simulink model "single_phase_ttype_inverter"  (R2026a)
settings: Solver=ode23tb  StopTime=simlength  FixedStep=tc  MaxStep=glb_time.tc
values from neighbouring files (symbols this model uses):
  afe_ctrl = param.afe.ctrl    [init_model.m]
  afe_pwm_phase_shift_mod1 = param.afe.behav.pwm_phase_shift_mod1    [init_model.m]
  DThs_init = param.thermal.DThs_init    [init_model.m]
  filters = param.ctrl.filters    [init_model.m]
  frt_data = param.frt.data    [init_model.m]
  glb_time = param.glb_time    [init_model.m]
  grid_emu = param.grid.emu    [init_model.m]
  kepsilon = param.spinv.kepsilon    [init_model.m]
  kp_align = param.ctrl.kp_align    [init_model.m]
  lim_down_align = param.ctrl.lim_down_align    [init_model.m]
  lim_up_align = param.ctrl.lim_up_align    [init_model.m]
  mavarage_filter_frequency_base_order = param.ctrl.mavarage_filter_frequency_base_order    [init_model.m]
  omega_set = param.spinv.omega_set    [init_model.m]
  single_phase_inverter_ctrl = param.spinv.ctrl    [init_model.m]
  Tambient = param.thermal.Tambient    [init_model.m]
  time_aux_power_supply_fault = param.sim.time_aux_power_supply_fault    [init_model.m]
  time_step_ref_1 = param.spinv.ref.time_step_ref_1    [init_model.m]
  time_step_ref_2 = param.spinv.ref.time_step_ref_2    [init_model.m]
  time_step_ref_3 = param.spinv.ref.time_step_ref_3    [init_model.m]
undefined symbols (not defined in the file or in its folder): delta_fht1, hwdata, ki_align, Ld_fht1, magnitude, omega_fht1, ts_inv, Vac_FS, Vdc_nom, Xbez
libraries: fl_lib x61, nesl_utility x39, moving_average_filter x11, moving_average_filter_cc x8, discrete_time_low_pass_filter x4, sl_discontinuities x3, single_phase_transformer_lib x3, linear_double_integrator_observer_ccaller x2, phase_shift_filter_ccaller x2, threephase_inductor_lib x1, dclink_for_two_levels x1, three_phase_pwm_modulator x1
(part 8 of 9)

== system single_phase_ttype_inverter/afe/AFE_control/afe_control/grid_voltage_phase_lock_loops/dq_pll/pll_stageB/double_integrator_observer ==
  phase : Inport
  Gain : Gain  Gain=afe_ctrl.di_obs.Ldso  Multiplication=Matrix(K*u)
  Gain1 : Gain  Gain=afe_ctrl.di_obs.Adso  Multiplication=Matrix(K*u)
  Gain2 : Gain  Gain=afe_ctrl.di_obs.Cso  Multiplication=Matrix(K*u)
  Selector : Selector  InputPortWidth=2  IndexOptions=Index vector (dialog)  Indices=2  OutputSizes=1
  Sum : Sum  Inputs=-+|
  Sum1 : Sum  Inputs=|++
  Unit Delay : UnitDelay  SampleTime=-1
  bounder1 : MATLAB Function  TreatAsAtomicUnit=on
  bounder2 : MATLAB Function  TreatAsAtomicUnit=on
  omega_hat : Outport
  wires:
  Gain/1 -> Sum1/1
  Selector/1 -> omega_hat/1
  Gain2/1 -> bounder2/1(u)  "theta_hat"
  Gain1/1 -> Sum1/2
  Sum1/1 -> Unit Delay/1
  Sum/1 -> bounder1/1(u)  "e"
  Unit Delay/1 -> Gain1/1, Selector/1, Gain2/1
  phase/1 -> Sum/2  "phase"
  bounder1/1(y) -> Gain/1  "e_bounded"
  bounder2/1(y) -> Sum/1  "theta_hat_bounded"

== system single_phase_ttype_inverter/afe/AFE_control/afe_control/grid_voltage_phase_lock_loops/dq_pll/pll_stageB/scheduled-p-gain ==
  In1 : Inport
  Switch : Switch  Criteria=u2 > Threshold  Threshold=0.5  SaturateOnIntegerOverflow=off  InputSameDT=off
  kp1 : Gain  Gain=afe_ctrl.pll_p  SaturateOnIntegerOverflow=on  OutDataTypeStr=Inherit: Same as input  ParamDataTypeStr=Inherit: Same as input
  kp3 : Gain  Gain=afe_ctrl.pll_p_frt  SaturateOnIntegerOverflow=on  OutDataTypeStr=Inherit: Same as input  ParamDataTypeStr=Inherit: Same as input
  Out2 : Outport
  wires:
  kp3/1 -> Switch/1
  kp1/1 -> Switch/3
  [frt_active_mod1] -> Switch/2
  In1/1 -> kp1/1, kp3/1
  Switch/1 -> Out2/1

== system single_phase_ttype_inverter/single_phase_inverter/single phase inverter control/single_phase_inverter_ctrl/single_phase_current_control/dqpi_current_controller/dq_vector_pi_ccaller/Reset ==
  Step : Step  Time=0.05  InitialValue=1  FinalValue=0
  en : Outport
  wires:
  Step/1 -> en/1

== system single_phase_ttype_inverter/single_phase_inverter/single phase inverter control/single_phase_inverter_ctrl/single_phase_current_control/dqpi_current_controller/i2alphabeta/first_harmonic_tracker ==
  u : Inport
  Bus Selector : BusSelector  OutputSignals=output_pu_hat,output_pu_hat_dot
  Constant1 : Constant  Value=6
  Constant2 : Constant  Value=glb_time.ts_inv
  Constant3 : Constant  Value=single_phase_inverter_ctrl.fht_load.omega_fht
  Constant4 : Constant  Value=single_phase_inverter_ctrl.fht_load.delta_fht
  Constant5 : Constant  Value=single_phase_inverter_ctrl.fht_load.Ld_fht(1)
  Constant6 : Constant  Value=single_phase_inverter_ctrl.fht_load.Ld_fht(2)
  Data Type Conversion{1..2,6..9} (6 alike) : DataTypeConversion  OutDataTypeStr=single  SaturateOnIntegerOverflow=off  RndMeth=Floor
  Data Type Conversion10 : DataTypeConversion  OutDataTypeStr=double  SaturateOnIntegerOverflow=off  RndMeth=Floor
  Data Type Conversion3 : DataTypeConversion  OutDataTypeStr=uint8  SaturateOnIntegerOverflow=off  RndMeth=Floor
  Data Type Conversion4 : DataTypeConversion  OutDataTypeStr=double  SaturateOnIntegerOverflow=off  RndMeth=Floor
  Data Type Conversion5 : DataTypeConversion  OutDataTypeStr=uint8  SaturateOnIntegerOverflow=off  RndMeth=Floor
  Gain : Gain  Gain=-1/single_phase_inverter_ctrl.fht_load.omega_fht
  Step : Step  Time=0.0125  InitialValue=1  FinalValue=0
  first_harmonic_tracker : CCaller  FunctionName=first_harmonic_tracker_process_simulink  PortSpecificationStruct="%)30     .    B \\   8    (     @         %    \"     D    !     0         %  0 \"0    $    _    07)G3F%M90  4&]R=$YA;64 4V-O<&4     26YD97@     5'EP90      4VEZ90      27-';&]B86P   X    P    !@    @    $          4    (     0    ,    !         !   P!O=70 #@   #     &    \"     0         !0    @    !     P    $         $  # &]U=  .    .     8    (    !          %    \"     $    &     0         0  ...(+4988 chars)"
  alpha : Outport
  beta : Outport  Port=2
  wires:
  Data Type Conversion4/1 -> alpha/1
  Data Type Conversion3/1 -> first_harmonic_tracker/1
  Data Type Conversion1/1 -> first_harmonic_tracker/3
  Data Type Conversion2/1 -> first_harmonic_tracker/2
  first_harmonic_tracker/1 -> Bus Selector/1
  Bus Selector/1 -> Data Type Conversion4/1  "<output_pu_hat>"
  Step/1 -> Data Type Conversion3/1
  u/1 -> Data Type Conversion2/1
  Constant2/1 -> Data Type Conversion1/1
  Constant1/1 -> Data Type Conversion5/1
  Data Type Conversion5/1 -> first_harmonic_tracker/8
  Constant3/1 -> Data Type Conversion6/1
  Data Type Conversion6/1 -> first_harmonic_tracker/4
  Constant4/1 -> Data Type Conversion7/1
  Data Type Conversion7/1 -> first_harmonic_tracker/5
  Constant5/1 -> Data Type Conversion8/1
  Data Type Conversion8/1 -> first_harmonic_tracker/6
  Constant6/1 -> Data Type Conversion9/1
  Data Type Conversion9/1 -> first_harmonic_tracker/7
  Bus Selector/2 -> Data Type Conversion10/1  "<output_pu_hat_dot>"
  Data Type Conversion10/1 -> Gain/1
  Gain/1 -> beta/1

== system single_phase_ttype_inverter/single_phase_inverter/single phase inverter control/single_phase_inverter_ctrl/single_phase_current_control/dqpi_current_controller/i2alphabeta/phase_shift_method ==
  i_alpha : Inport
  Gain : Gain  Gain=-1
  phase shift filter : phase_shift_filter/phase shift filter  f=frequency_set  scaling_factor=1  ts=glb_time.ts_inv
  i_alpha_phase_shift_m : Outport
  i_beta_phase_shift_m : Outport  Port=2
  wires:
  i_alpha/1 -> phase shift filter/1, i_alpha_phase_shift_m/1
  Gain/1 -> i_beta_phase_shift_m/1  "i_beta_phase_shift_methos"
  phase shift filter/1 -> Gain/1

== system single_phase_ttype_inverter/single_phase_inverter/single phase inverter control/single_phase_inverter_ctrl/single_phase_current_control/dqpi_current_controller/i2alphabeta/phase_shift_method_ccaller ==
  i_alpha : Inport
  Gain : Gain  Gain=-1
  phase_shift_filter_ccaller : phase_shift_filter_ccaller/phase_shift_filter_ccaller  freq_m=frequency_set  ts_m=glb_time.ts_inv  scaling_m=1  reset_time_release=0.025  instance=0  tc_m=-1
  i_alpha_phase_shift_m : Outport
  i_beta_phase_shift_m : Outport  Port=2
  wires:
  phase_shift_filter_ccaller/1 -> Gain/1
  Gain/1 -> i_beta_phase_shift_m/1  "i_beta_phase_shift_methos"
  i_alpha/1 -> i_alpha_phase_shift_m/1, phase_shift_filter_ccaller/1

== system single_phase_ttype_inverter/single_phase_inverter/single phase inverter control/single_phase_inverter_ctrl/single_phase_current_control/dqpi_current_controller/i2alphabeta/sogi ==
  u : Inport
  Constant2 : Constant  Value=omega_set
  Product : Product
  Product1 : Product
  Sum1 : Sum  Inputs=|+-
  Sum3 : Sum  Inputs=-+|
  integrator_1 : Subsystem
  integrator_2 : Subsystem
  kepsilon : Gain  Gain=kepsilon
  ualpha : Outport
  ubeta : Outport  Port=2
  wires:
  u/1 -> ualpha/1, Sum3/2
  Sum3/1 -> kepsilon/1
  kepsilon/1 -> Sum1/1
  Sum1/1 -> Product/2
  Product/1 -> integrator_1/1(in)
  integrator_1/1(out) -> Product1/2, Sum3/1
  Constant2/1 -> Product/1, Product1/1
  Product1/1 -> integrator_2/1(in)
  integrator_2/1(out) -> ubeta/1, Sum1/2

== system single_phase_ttype_inverter/single_phase_inverter/single phase inverter control/single_phase_inverter_ctrl/single_phase_current_control/dqpi_current_controller/i2alphabeta/sogi_ccaller ==
  input : Inport
  Bus Selector : BusSelector  OutputSignals=sogi_flt_output_alpha,sogi_flt_output_beta
  CCaller : CCaller  FunctionName=sogi_flt_process_simulink  PortSpecificationStruct="%)30     .    . P   8    (     @         %    \"     <    !     0         %  0 \"0    $    _    07)G3F%M90  4&]R=$YA;64 4V-O<&4     26YD97@     5'EP90      4VEZ90      27-';&]B86P   X    P    !@    @    $          4    (     0    ,    !         !   P!O=70 #@   #     &    \"     0         !0    @    !     P    $         $  # &]U=  .    .     8    (    !          %    \"     $    &     0         0   ...(+3829 chars)"
  Constant1 : Constant  Value=glb_time.ts_inv
  Constant2 : Constant  Value=omega_set
  Constant3 : Constant  Value=kepsilon
  Constant4 : Constant  Value=2
  Data Type Conversion{1..2,4,6} (4 alike) : DataTypeConversion  OutDataTypeStr=single  SaturateOnIntegerOverflow=off  RndMeth=Floor
  Data Type Conversion3 : DataTypeConversion  OutDataTypeStr=uint8  SaturateOnIntegerOverflow=off  RndMeth=Floor
  Data Type Conversion5 : DataTypeConversion  OutDataTypeStr=double  SaturateOnIntegerOverflow=off  RndMeth=Floor
  Data Type Conversion7 : DataTypeConversion  OutDataTypeStr=double  SaturateOnIntegerOverflow=off  RndMeth=Floor
  Data Type Conversion8 : DataTypeConversion  OutDataTypeStr=uint8  SaturateOnIntegerOverflow=off  RndMeth=Floor
  Reset : Subsystem
  Terminator : Terminator
  Zero-Order Hold{1..6} (6 alike) : ZeroOrderHold  SampleTime=-1
  alpha : Outport
  beta : Outport  Port=2
  wires:
  Zero-Order Hold6/1 -> Data Type Conversion4/1
  Data Type Conversion4/1 -> CCaller/1
  Bus Selector/1 -> Data Type Conversion7/1  "<sogi_flt_output_alpha>"
  CCaller/1 -> Bus Selector/1
  Constant4/1 -> Zero-Order Hold5/1
  Zero-Order Hold5/1 -> Data Type Conversion3/1
  Constant2/1 -> Zero-Order Hold1/1
  Zero-Order Hold1/1 -> Data Type Conversion2/1
  Zero-Order Hold2/1 -> Data Type Conversion1/1
  Constant1/1 -> Zero-Order Hold2/1
  Reset/1(en) -> Zero-Order Hold4/1
  Zero-Order Hold4/1 -> Data Type Conversion8/1
  input/1 -> alpha/1, Zero-Order Hold6/1
  Bus Selector/2 -> Data Type Conversion5/1  "<sogi_flt_output_beta>"
  Data Type Conversion5/1 -> beta/1
  Data Type Conversion3/1 -> CCaller/6
  Data Type Conversion8/1 -> CCaller/5
  Data Type Conversion2/1 -> CCaller/3
  Data Type Conversion1/1 -> CCaller/2
  Data Type Conversion6/1 -> CCaller/4
  Zero-Order Hold3/1 -> Data Type Conversion6/1
  Constant3/1 -> Zero-Order Hold3/1
  Data Type Conversion7/1 -> Terminator/1

== system single_phase_ttype_inverter/single_phase_inverter/single phase inverter control/single_phase_inverter_ctrl/sistem_identification/open loop u//f/sogi_ccaller/Reset ==
  Step : Step  Time=0.025  InitialValue=1  FinalValue=0
  en : Outport
  wires:
  Step/1 -> en/1

== system single_phase_ttype_inverter/afe/AFE_control/afe_control/grid_voltage_phase_lock_loops/DDSRF-PLL/pll_stageA/filter_and_transformation/first_harmonic_tracker_phase_u ==
  u : Inport
  Bus Selector : BusSelector  OutputSignals=output_pu_hat
  C Caller : CCaller  FunctionName=first_harmonic_tracker_process_simulink  PortSpecificationStruct="%)30     .    B \\   8    (     @         %    \"     D    !     0         %  0 \"0    $    _    07)G3F%M90  4&]R=$YA;64 4V-O<&4     26YD97@     5'EP90      4VEZ90      27-';&]B86P   X    P    !@    @    $          4    (     0    ,    !         !   P!O=70 #@   #     &    \"     0         !0    @    !     P    $         $  # &]U=  .    .     8    (    !          %    \"     $    &     0         0  ...(+4988 chars)"
  Constant : Constant  Value=glb_time.ts_afe
  Constant1 : Constant  Value=6
  Constant4 : Constant  Value=afe_ctrl.fht_grid.omega_fht
  Constant5 : Constant  Value=afe_ctrl.fht_grid.delta_fht
  Constant6 : Constant  Value=afe_ctrl.fht_grid.Ld_fht(1)
  Constant7 : Constant  Value=afe_ctrl.fht_grid.Ld_fht(2)
  Data Type Conversion{1..2,6..9} (6 alike) : DataTypeConversion  OutDataTypeStr=single  SaturateOnIntegerOverflow=off  RndMeth=Floor
  Data Type Conversion3 : DataTypeConversion  OutDataTypeStr=uint8  SaturateOnIntegerOverflow=off  RndMeth=Floor
  Data Type Conversion4 : DataTypeConversion  OutDataTypeStr=double  SaturateOnIntegerOverflow=off  RndMeth=Floor
  Data Type Conversion5 : DataTypeConversion  OutDataTypeStr=uint8  SaturateOnIntegerOverflow=off  RndMeth=Floor
  Step : Step  Time=0.0125  InitialValue=1  FinalValue=0
  u_hat : Outport
  wires:
  Data Type Conversion4/1 -> u_hat/1
  Data Type Conversion3/1 -> C Caller/1
  Data Type Conversion1/1 -> C Caller/3
  Data Type Conversion2/1 -> C Caller/2
  C Caller/1 -> Bus Selector/1
  Bus Selector/1 -> Data Type Conversion4/1  "<output_pu_hat>"
  Step/1 -> Data Type Conversion3/1
  u/1 -> Data Type Conversion2/1
  Constant/1 -> Data Type Conversion1/1
  Constant1/1 -> Data Type Conversion5/1
  Constant4/1 -> Data Type Conversion6/1
  Constant6/1 -> Data Type Conversion8/1
  Constant7/1 -> Data Type Conversion9/1
  Constant5/1 -> Data Type Conversion7/1
  Data Type Conversion5/1 -> C Caller/8
  Data Type Conversion6/1 -> C Caller/4
  Data Type Conversion7/1 -> C Caller/5
  Data Type Conversion8/1 -> C Caller/6
  Data Type Conversion9/1 -> C Caller/7

== system single_phase_ttype_inverter/afe/AFE_control/afe_control/grid_voltage_phase_lock_loops/DDSRF-PLL/pll_stageA/filter_and_transformation/first_harmonic_tracker_phase_v ==
  u : Inport
  Bus Selector : BusSelector  OutputSignals=output_pu_hat
  C Caller : CCaller  FunctionName=first_harmonic_tracker_process_simulink  PortSpecificationStruct="%)30     .    B \\   8    (     @         %    \"     D    !     0         %  0 \"0    $    _    07)G3F%M90  4&]R=$YA;64 4V-O<&4     26YD97@     5'EP90      4VEZ90      27-';&]B86P   X    P    !@    @    $          4    (     0    ,    !         !   P!O=70 #@   #     &    \"     0         !0    @    !     P    $         $  # &]U=  .    .     8    (    !          %    \"     $    &     0         0  ...(+4988 chars)"
  Constant : Constant  Value=glb_time.ts_afe
  Constant1 : Constant  Value=8
  Constant4 : Constant  Value=afe_ctrl.fht_grid.omega_fht
  Constant5 : Constant  Value=afe_ctrl.fht_grid.delta_fht
  Constant6 : Constant  Value=afe_ctrl.fht_grid.Ld_fht(1)
  Constant7 : Constant  Value=afe_ctrl.fht_grid.Ld_fht(2)
  Data Type Conversion{1..2,6..9} (6 alike) : DataTypeConversion  OutDataTypeStr=single  SaturateOnIntegerOverflow=off  RndMeth=Floor
  Data Type Conversion3 : DataTypeConversion  OutDataTypeStr=uint8  SaturateOnIntegerOverflow=off  RndMeth=Floor
  Data Type Conversion4 : DataTypeConversion  OutDataTypeStr=double  SaturateOnIntegerOverflow=off  RndMeth=Floor
  Data Type Conversion5 : DataTypeConversion  OutDataTypeStr=uint8  SaturateOnIntegerOverflow=off  RndMeth=Floor
  Step : Step  Time=0.0125  InitialValue=1  FinalValue=0
  u_hat : Outport
  wires:
  Data Type Conversion9/1 -> C Caller/7
  Data Type Conversion8/1 -> C Caller/6
  Data Type Conversion7/1 -> C Caller/5
  Data Type Conversion6/1 -> C Caller/4
  Data Type Conversion5/1 -> C Caller/8
  Constant5/1 -> Data Type Conversion7/1
  Constant7/1 -> Data Type Conversion9/1
  Constant6/1 -> Data Type Conversion8/1
  Constant4/1 -> Data Type Conversion6/1
  Constant1/1 -> Data Type Conversion5/1
  Constant/1 -> Data Type Conversion1/1
  u/1 -> Data Type Conversion2/1
  Step/1 -> Data Type Conversion3/1
  Bus Selector/1 -> Data Type Conversion4/1  "<output_pu_hat>"
  C Caller/1 -> Bus Selector/1
  Data Type Conversion2/1 -> C Caller/2
  Data Type Conversion1/1 -> C Caller/3
  Data Type Conversion3/1 -> C Caller/1
  Data Type Conversion4/1 -> u_hat/1

== system single_phase_ttype_inverter/afe/AFE_control/afe_control/grid_voltage_phase_lock_loops/DDSRF-PLL/pll_stageA/filter_and_transformation/first_harmonic_tracker_phase_w ==
  u : Inport
  Bus Selector : BusSelector  OutputSignals=output_pu_hat
  C Caller : CCaller  FunctionName=first_harmonic_tracker_process_simulink  PortSpecificationStruct="%)30     .    B \\   8    (     @         %    \"     D    !     0         %  0 \"0    $    _    07)G3F%M90  4&]R=$YA;64 4V-O<&4     26YD97@     5'EP90      4VEZ90      27-';&]B86P   X    P    !@    @    $          4    (     0    ,    !         !   P!O=70 #@   #     &    \"     0         !0    @    !     P    $         $  # &]U=  .    .     8    (    !          %    \"     $    &     0         0  ...(+4988 chars)"
  Constant : Constant  Value=glb_time.ts_afe
  Constant1 : Constant  Value=10
  Constant4 : Constant  Value=afe_ctrl.fht_grid.omega_fht
  Constant5 : Constant  Value=afe_ctrl.fht_grid.delta_fht
  Constant6 : Constant  Value=afe_ctrl.fht_grid.Ld_fht(1)
  Constant7 : Constant  Value=afe_ctrl.fht_grid.Ld_fht(2)
  Data Type Conversion{1..2,6..9} (6 alike) : DataTypeConversion  OutDataTypeStr=single  SaturateOnIntegerOverflow=off  RndMeth=Floor
  Data Type Conversion3 : DataTypeConversion  OutDataTypeStr=uint8  SaturateOnIntegerOverflow=off  RndMeth=Floor
  Data Type Conversion4 : DataTypeConversion  OutDataTypeStr=double  SaturateOnIntegerOverflow=off  RndMeth=Floor
  Data Type Conversion5 : DataTypeConversion  OutDataTypeStr=uint8  SaturateOnIntegerOverflow=off  RndMeth=Floor
  Step : Step  Time=0.0125  InitialValue=1  FinalValue=0
  u_hat : Outport
  wires:
  Data Type Conversion4/1 -> u_hat/1
  Data Type Conversion3/1 -> C Caller/1
  Data Type Conversion1/1 -> C Caller/3
  Data Type Conversion2/1 -> C Caller/2
  C Caller/1 -> Bus Selector/1
  Bus Selector/1 -> Data Type Conversion4/1  "<output_pu_hat>"
  Step/1 -> Data Type Conversion3/1
  u/1 -> Data Type Conversion2/1
  Constant/1 -> Data Type Conversion1/1
  Constant1/1 -> Data Type Conversion5/1
  Constant4/1 -> Data Type Conversion6/1
  Constant6/1 -> Data Type Conversion8/1
  Constant7/1 -> Data Type Conversion9/1
  Constant5/1 -> Data Type Conversion7/1
  Data Type Conversion5/1 -> C Caller/8
  Data Type Conversion6/1 -> C Caller/4
  Data Type Conversion7/1 -> C Caller/5
  Data Type Conversion8/1 -> C Caller/6
  Data Type Conversion9/1 -> C Caller/7

== system single_phase_ttype_inverter/afe/AFE_control/afe_control/grid_voltage_phase_lock_loops/DDSRF-PLL/pll_stageA/sequences/ddsrf ==
  u_grid_alpha : Inport
  u_grid_beta : Inport  Port=2
  phase_angle : Inport  Port=3
  Gain : Gain  Gain=2
  Sum : Sum  Inputs=|+-
  Sum1 : Sum  Inputs=|+-
  Sum2 : Sum  Inputs=-+|
  Sum3 : Sum  Inputs=-+|
  alphabeta2xieta_neg : MATLAB Function  TreatAsAtomicUnit=on
  alphabeta2xieta_neg1 : MATLAB Function  TreatAsAtomicUnit=on
  alphabeta2xieta_pos : MATLAB Function  TreatAsAtomicUnit=on
  alphabeta2xieta_pos1 : MATLAB Function  TreatAsAtomicUnit=on
  bounder2 : MATLAB Function  TreatAsAtomicUnit=on
  discrete-time-low-pass-filter{,1..3} (4 alike) : discrete_time_low_pass_filter/discrete-time-low-pass-filter  tau=afe_ctrl.tau_ddsrf  ts=glb_time.ts_afe
  u_grid_pos_xi : Outport
  u_grid_pos_eta : Outport  Port=2
  u_grid_neg_xi : Outport  Port=3
  u_grid_neg_eta : Outport  Port=4
  wires:
  phase_angle/1 -> alphabeta2xieta_pos/3(gamma), alphabeta2xieta_neg/3(gamma), Gain/1  "phase_angle"
  u_grid_beta/1 -> alphabeta2xieta_pos/2(beta), alphabeta2xieta_neg/2(beta)  "u_grid_beta"
  u_grid_alpha/1 -> alphabeta2xieta_pos/1(alpha), alphabeta2xieta_neg/1(alpha)  "u_grid_alpha"
  alphabeta2xieta_pos/1(xi) -> Sum/1  "u_grid_pos_xi"
  Sum/1 -> discrete-time-low-pass-filter/1
  alphabeta2xieta_pos/2(eta) -> Sum1/1  "u_grid_pos_eta"
  Sum1/1 -> discrete-time-low-pass-filter1/1
  alphabeta2xieta_neg/1(xi) -> Sum2/2  "u_grid_neg_xi"
  Sum2/1 -> discrete-time-low-pass-filter2/1
  Sum3/1 -> discrete-time-low-pass-filter3/1
  alphabeta2xieta_neg/2(eta) -> Sum3/2  "u_grid_neg_eta"
  Gain/1 -> bounder2/1(u)
  discrete-time-low-pass-filter/1 -> u_grid_pos_xi/1, alphabeta2xieta_neg1/1(alpha)
  discrete-time-low-pass-filter1/1 -> u_grid_pos_eta/1, alphabeta2xieta_neg1/2(beta)
  discrete-time-low-pass-filter2/1 -> u_grid_neg_xi/1, alphabeta2xieta_pos1/1(alpha)
  discrete-time-low-pass-filter3/1 -> u_grid_neg_eta/1, alphabeta2xieta_pos1/2(beta)
  bounder2/1(y) -> [phase_angle_2]
  [phase_angle_2] -> alphabeta2xieta_pos1/3(gamma)
  [phase_angle_2] -> alphabeta2xieta_neg1/3(gamma)
  alphabeta2xieta_pos1/1(xi) -> Sum/2
  alphabeta2xieta_pos1/2(eta) -> Sum1/2
  alphabeta2xieta_neg1/1(xi) -> Sum2/1
  alphabeta2xieta_neg1/2(eta) -> Sum3/1
